simulink model "shashankfile"  (R2024a)
settings: Solver=VariableStepAuto  StartTime=0.0  StopTime=1  RelTol=1e-3
libraries: simulink_extras x1, cstblocks x1, dspobslib x1
settings Model: Creator=eniya  LastModifiedBy=SHASHANK DADURIA

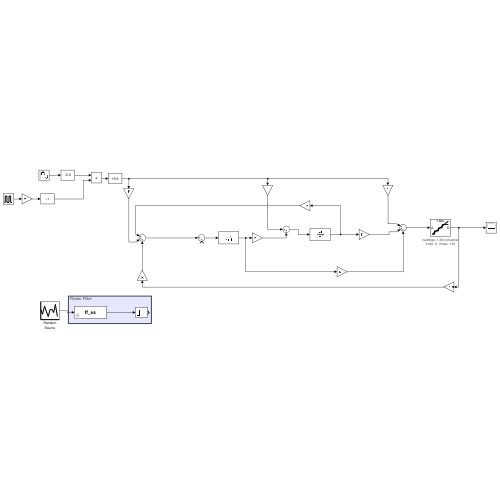
[thumbnail: Simulink's stored preview of the top-level diagram]
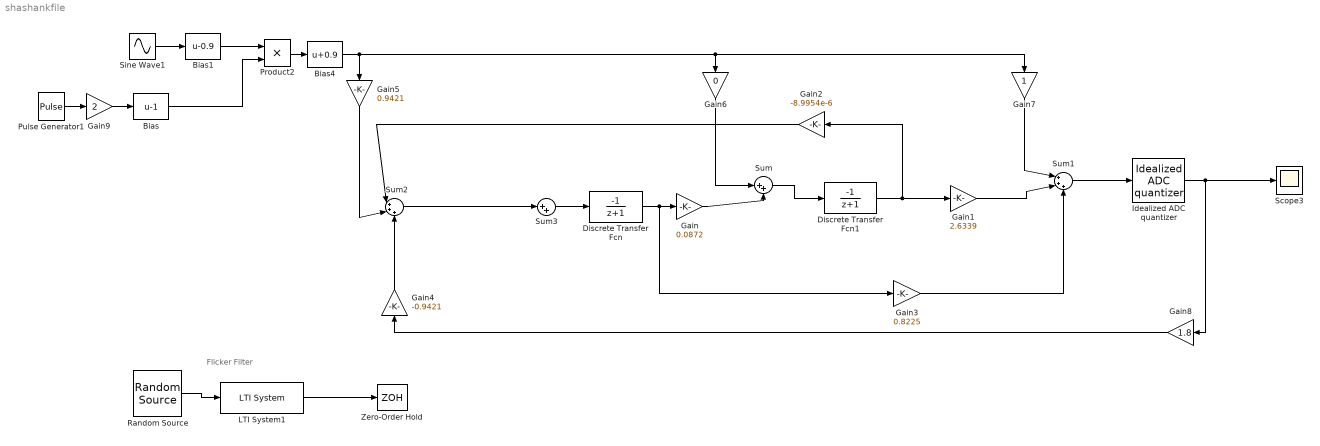
== system shashankfile ==
  note: Flicker Filter
  Bias : Bias  Bias=-1  SaturateOnIntegerOverflow=off
  Bias1 : Bias  Bias=-0.9  SaturateOnIntegerOverflow=off
  Bias4 : Bias  Bias=0.9  SaturateOnIntegerOverflow=off
  Discrete Transfer Fcn : DiscreteTransferFcn  Numerator=[-1]  Denominator=[1 1]
  Discrete Transfer Fcn1 : DiscreteTransferFcn  Numerator=[-1]  Denominator=[1 1]
  Gain : Gain  Gain=0.0872
  Gain1 : Gain  Gain=2.6339
  Gain2 : Gain  Gain=-8.9954e-6
  Gain3 : Gain  Gain=0.8225
  Gain4 : Gain  Gain=-0.9421
  Gain5 : Gain  Gain=0.9421
  Gain6 : Gain  Gain=0
  Gain7 : Gain
  Gain8 : Gain  Gain=1.8
  Gain9 : Gain  Gain=2
  Idealized ADC quantizer : simulink_extras/Additional Discrete/Idealized ADC quantizer  NumberOfConverterBits=1  Vmin=0  Vmax=1.8  OutputDataType=int16  OutputNegativeValues=off
  LTI System1 : cstblocks/LTI System  sys=ff_ss  IC=[]  PadeOrder=0
  Product2 : Product
  Pulse Generator1 : DiscretePulseGenerator  PulseType=Time based  Period=2/(2048000*4)  PulseWidth=50
  Random Source : dspobslib/Random Source  SrcType=Gaussian  NormMethod=Ziggurat  CltLength=12  MinVal=0  MaxVal=1  MeanVal=0  VarVal=1e-7  RepMode=Not repeatable  rawSeed=1  IsInherit=off  SampMode=Discrete  SampTime=1/(2000*4096)  SampFrame=1  DataType=Double  OutComplex=Real  OutputFrames=off
  Scope3 : Scope
  Sine Wave1 : Sin  Amplitude=0.5  Bias=0.9  Frequency=((2000*1024)*127*2*2*pi)/(32768*32)  SampleTime=1/(2e3*4096)
  Sum : Sum  Inputs=|++
  Sum1 : Sum  Inputs=|+++
  Sum2 : Sum  Inputs=|+++
  Sum3 : Sum  Inputs=|++
  Zero-Order Hold : ZeroOrderHold  SampleTime=1/(2000*4096)
  wires:
  Gain/1 -> Sum/2
  Gain5/1 -> Sum2/2
  Gain7/1 -> Sum1/1
  Gain1/1 -> Sum1/2
  Discrete Transfer Fcn1/1 -> Gain2/1, Gain1/1
  Gain2/1 -> Sum2/1
  Gain6/1 -> Sum/1
  Bias4/1 -> Gain7/1, Gain6/1, Gain5/1
  Sum/1 -> Discrete Transfer Fcn1/1
  Gain3/1 -> Sum1/3
  Gain4/1 -> Sum2/3
  Sum1/1 -> Idealized ADC quantizer/1
  Discrete Transfer Fcn/1 -> Gain3/1, Gain/1
  Idealized ADC quantizer/1 -> Scope3/1, Gain8/1
  Gain8/1 -> Gain4/1
  Bias/1 -> Product2/2
  Pulse Generator1/1 -> Gain9/1
  Gain9/1 -> Bias/1
  Bias1/1 -> Product2/1
  Product2/1 -> Bias4/1
  Sine Wave1/1 -> Bias1/1
  LTI System1/1 -> Zero-Order Hold/1
  Random Source/1 -> LTI System1/1
  Sum2/1 -> Sum3/1
  Sum3/1 -> Discrete Transfer Fcn/1
